simulink model "fft_biplex_real_4x_dsp48_opt_test"  (Simulink 7.4)
settings: Solver=VariableStepDiscrete  StartTime=0.0  StopTime=128  RelTol=1e-3
libraries: xbsIndex_r4 x620, casper_library_misc x24, casper_library_delays x6, casper_library_ffts_twiddle x1, simulink x1
(part 6 of 7)

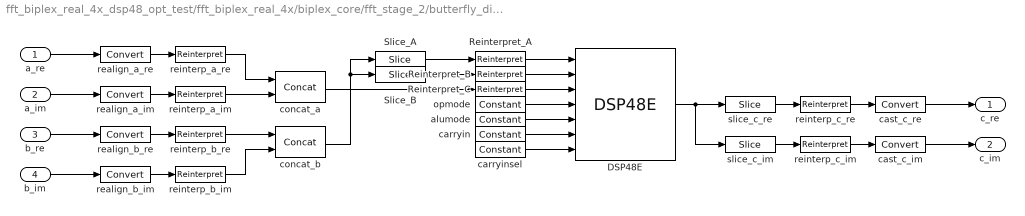
== system fft_biplex_real_4x_dsp48_opt_test/fft_biplex_real_4x/biplex_core/fft_stage_2/butterfly_direct/cadd ==
  a_re : Inport  OutDataType=sfix(16)  OutScaling=2^0
  a_im : Inport  Port=2  OutDataType=sfix(16)  OutScaling=2^0
  b_re : Inport  Port=3  OutDataType=sfix(16)  OutScaling=2^0
  b_im : Inport  Port=4  OutDataType=sfix(16)  OutScaling=2^0
  DSP48E : xbsIndex_r4/DSP48E  use_a=Direct from A Port  use_b=Direct from B Port  pattern_from_creg=off  pattern='000000000000'  mask_from_creg=off  pattern_mask='3FFFFFFFFFFF'  reset_preg=off  sel_rounding_mask=Select mask  use_op=off  use_creg=on  rst_all=off  en_all=off  use_pcin=off  use_carrycascin=off  use_multsignin=off  use_carryout=off  use_patterndetect=off  use_patternbdetect=off  use_overflow=off  use_underflow=off  use_acout=off  use_bcout=off  use_pcout=off  use_multsignout=off  use_carrycascout=off  pipeline_a=1  pipeline_b=1  pipeline_acout=1  pipeline_bcout=1  pipeline_c=on  pipeline_p=on  pipeline_mult=on  pipeline_opmode=on  pipeline_alumode=on  pipeline_carryin=on  pipeline_carryinsel=on  rst_a=off  rst_b=off  rst_c=off  rst_mult=off  rst_p=off  rst_carry_in=off  rst_alumode=off  rst_ctrl=off  en_a1=off  en_a2=off  en_b1=off  en_b2=off  en_c=off  en_mult=off  en_p=off  en_carry_in=off  en_alumode=off  en_multcarryin=off  en_ctrl=off  use_synth_model=off  addsub_mode=TWO24  xl_useadderonly=off  block_type=dsp48e
      settings: block_version=10.1.3
  Reinterpret_A : xbsIndex_r4/Reinterpret  force_arith_type=on  arith_type="Signed  (2's comp)"  force_bin_pt=on  bin_pt=0  block_type=reinterpret
      settings: infoedit="Changes signal type without altering the binary representation.   You can changed the signal between signed and unsigned, and relocate the binary point.<br><br>Hardware notes: In hardware this block costs nothing.<br><br>Example:  Suppose the input is 6 bits wide, signed, with 2 fractional bits, and the output is forced to unsigned with 0 fractional bits.  Then an input of -2.0 (1110.00 in binary 2's complement) becomes an output of 56 (111000 in binary)."  block_version=10.1.3
  Reinterpret_B : xbsIndex_r4/Reinterpret  force_arith_type=on  arith_type="Signed  (2's comp)"  force_bin_pt=on  bin_pt=0  block_type=reinterpret
      settings: infoedit="Changes signal type without altering the binary representation.   You can changed the signal between signed and unsigned, and relocate the binary point.<br><br>Hardware notes: In hardware this block costs nothing.<br><br>Example:  Suppose the input is 6 bits wide, signed, with 2 fractional bits, and the output is forced to unsigned with 0 fractional bits.  Then an input of -2.0 (1110.00 in binary 2's complement) becomes an output of 56 (111000 in binary)."  block_version=10.1.3
  Reinterpret_C : xbsIndex_r4/Reinterpret  force_arith_type=on  arith_type="Signed  (2's comp)"  force_bin_pt=on  bin_pt=0  block_type=reinterpret
      settings: infoedit="Changes signal type without altering the binary representation.   You can changed the signal between signed and unsigned, and relocate the binary point.<br><br>Hardware notes: In hardware this block costs nothing.<br><br>Example:  Suppose the input is 6 bits wide, signed, with 2 fractional bits, and the output is forced to unsigned with 0 fractional bits.  Then an input of -2.0 (1110.00 in binary 2's complement) becomes an output of 56 (111000 in binary)."  block_version=10.1.3
  Slice_A : xbsIndex_r4/Slice  nbits=30  boolean_output=off  mode=Upper Bit Location + Width  bit1=0  base1=MSB of Input  bit0=0  base0=LSB of Input  dbl_ovrd=off  block_type=slice
  Slice_B : xbsIndex_r4/Slice  nbits=18  boolean_output=off  mode=Lower Bit Location + Width  bit1=0  base1=MSB of Input  bit0=0  base0=LSB of Input  dbl_ovrd=off  block_type=slice
  alumode : xbsIndex_r4/Constant  arith_type=Unsigned  const=0  n_bits=4  bin_pt=0  explicit_period=off  period=1  equ=P=C  opselect=C  inp2=PCIN>>17  opr=+  inp1=P  carry=CIN  dbl_ovrd=off  block_type=constant
  carryin : xbsIndex_r4/Constant  arith_type=Unsigned  const=0  n_bits=1  bin_pt=0  explicit_period=off  period=1  equ=P=C  opselect=C  inp2=PCIN>>17  opr=+  inp1=P  carry=CIN  dbl_ovrd=off  block_type=constant
  carryinsel : xbsIndex_r4/Constant  arith_type=Unsigned  const=0  n_bits=3  bin_pt=0  explicit_period=off  period=1  equ=P=C  opselect=C  inp2=PCIN>>17  opr=+  inp1=P  carry=CIN  dbl_ovrd=off  block_type=constant
  cast_c_im : xbsIndex_r4/Convert  arith_type="Signed  (2's comp)"  n_bits=9  bin_pt=7  quantization=Truncate  overflow=Wrap  latency=0  dbl_ovrd=off  pipeline=on  block_type=convert
      settings: block_version=10.1.3
  cast_c_re : xbsIndex_r4/Convert  arith_type="Signed  (2's comp)"  n_bits=9  bin_pt=7  quantization=Truncate  overflow=Wrap  latency=0  dbl_ovrd=off  pipeline=on  block_type=convert
      settings: block_version=10.1.3
  concat_a : xbsIndex_r4/Concat  num_inputs=2  dbl_ovrd=off  block_type=concat
  concat_b : xbsIndex_r4/Concat  num_inputs=2  dbl_ovrd=off  block_type=concat
  opmode : xbsIndex_r4/Constant  arith_type=Unsigned  const=51  n_bits=7  bin_pt=0  explicit_period=off  period=1  equ=P=C  opselect=C  inp2=PCIN>>17  opr=+  inp1=P  carry=CIN  dbl_ovrd=off  block_type=constant
  realign_a_im : xbsIndex_r4/Convert  arith_type="Signed  (2's comp)"  n_bits=24  bin_pt=22  quantization=Truncate  overflow=Wrap  latency=0  dbl_ovrd=off  pipeline=on  block_type=convert
      settings: block_version=10.1.3
  realign_a_re : xbsIndex_r4/Convert  arith_type="Signed  (2's comp)"  n_bits=24  bin_pt=22  quantization=Truncate  overflow=Wrap  latency=0  dbl_ovrd=off  pipeline=on  block_type=convert
      settings: block_version=10.1.3
  realign_b_im : xbsIndex_r4/Convert  arith_type="Signed  (2's comp)"  n_bits=24  bin_pt=22  quantization=Truncate  overflow=Wrap  latency=0  dbl_ovrd=off  pipeline=on  block_type=convert
      settings: block_version=10.1.3
  realign_b_re : xbsIndex_r4/Convert  arith_type="Signed  (2's comp)"  n_bits=24  bin_pt=22  quantization=Truncate  overflow=Wrap  latency=0  dbl_ovrd=off  pipeline=on  block_type=convert
      settings: block_version=10.1.3
  reinterp_a_im : xbsIndex_r4/Reinterpret  force_arith_type=on  arith_type=Unsigned  force_bin_pt=on  bin_pt=0  block_type=reinterpret
      settings: infoedit="Changes signal type without altering the binary representation.   You can changed the signal between signed and unsigned, and relocate the binary point.<br><br>Hardware notes: In hardware this block costs nothing.<br><br>Example:  Suppose the input is 6 bits wide, signed, with 2 fractional bits, and the output is forced to unsigned with 0 fractional bits.  Then an input of -2.0 (1110.00 in binary 2's complement) becomes an output of 56 (111000 in binary)."  block_version=10.1.3
  reinterp_a_re : xbsIndex_r4/Reinterpret  force_arith_type=on  arith_type=Unsigned  force_bin_pt=on  bin_pt=0  block_type=reinterpret
      settings: infoedit="Changes signal type without altering the binary representation.   You can changed the signal between signed and unsigned, and relocate the binary point.<br><br>Hardware notes: In hardware this block costs nothing.<br><br>Example:  Suppose the input is 6 bits wide, signed, with 2 fractional bits, and the output is forced to unsigned with 0 fractional bits.  Then an input of -2.0 (1110.00 in binary 2's complement) becomes an output of 56 (111000 in binary)."  block_version=10.1.3
  reinterp_b_im : xbsIndex_r4/Reinterpret  force_arith_type=on  arith_type=Unsigned  force_bin_pt=on  bin_pt=0  block_type=reinterpret
      settings: infoedit="Changes signal type without altering the binary representation.   You can changed the signal between signed and unsigned, and relocate the binary point.<br><br>Hardware notes: In hardware this block costs nothing.<br><br>Example:  Suppose the input is 6 bits wide, signed, with 2 fractional bits, and the output is forced to unsigned with 0 fractional bits.  Then an input of -2.0 (1110.00 in binary 2's complement) becomes an output of 56 (111000 in binary)."  block_version=10.1.3
  reinterp_b_re : xbsIndex_r4/Reinterpret  force_arith_type=on  arith_type=Unsigned  force_bin_pt=on  bin_pt=0  block_type=reinterpret
      settings: infoedit="Changes signal type without altering the binary representation.   You can changed the signal between signed and unsigned, and relocate the binary point.<br><br>Hardware notes: In hardware this block costs nothing.<br><br>Example:  Suppose the input is 6 bits wide, signed, with 2 fractional bits, and the output is forced to unsigned with 0 fractional bits.  Then an input of -2.0 (1110.00 in binary 2's complement) becomes an output of 56 (111000 in binary)."  block_version=10.1.3
  reinterp_c_im : xbsIndex_r4/Reinterpret  force_arith_type=on  arith_type="Signed  (2's comp)"  force_bin_pt=on  bin_pt=22  block_type=reinterpret
      settings: infoedit="Changes signal type without altering the binary representation.   You can changed the signal between signed and unsigned, and relocate the binary point.<br><br>Hardware notes: In hardware this block costs nothing.<br><br>Example:  Suppose the input is 6 bits wide, signed, with 2 fractional bits, and the output is forced to unsigned with 0 fractional bits.  Then an input of -2.0 (1110.00 in binary 2's complement) becomes an output of 56 (111000 in binary)."  block_version=10.1.3
  reinterp_c_re : xbsIndex_r4/Reinterpret  force_arith_type=on  arith_type="Signed  (2's comp)"  force_bin_pt=on  bin_pt=22  block_type=reinterpret
      settings: infoedit="Changes signal type without altering the binary representation.   You can changed the signal between signed and unsigned, and relocate the binary point.<br><br>Hardware notes: In hardware this block costs nothing.<br><br>Example:  Suppose the input is 6 bits wide, signed, with 2 fractional bits, and the output is forced to unsigned with 0 fractional bits.  Then an input of -2.0 (1110.00 in binary 2's complement) becomes an output of 56 (111000 in binary)."  block_version=10.1.3
  slice_c_im : xbsIndex_r4/Slice  nbits=24  boolean_output=off  mode=Lower Bit Location + Width  bit1=0  base1=MSB of Input  bit0=0  base0=LSB of Input  dbl_ovrd=off  block_type=slice
  slice_c_re : xbsIndex_r4/Slice  nbits=24  boolean_output=off  mode=Lower Bit Location + Width  bit1=0  base1=MSB of Input  bit0=24  base0=LSB of Input  dbl_ovrd=off  block_type=slice
  c_re : Outport  OutDataType=sfix(16)  OutScaling=2^0
  c_im : Outport  Port=2  OutDataType=sfix(16)  OutScaling=2^0
  wires:
  realign_b_im/1 -> reinterp_b_im/1
  realign_b_re/1 -> reinterp_b_re/1
  realign_a_im/1 -> reinterp_a_im/1
  realign_a_re/1 -> reinterp_a_re/1
  a_re/1 -> realign_a_re/1
  b_re/1 -> realign_b_re/1
  Reinterpret_A/1 -> DSP48E/1
  Reinterpret_B/1 -> DSP48E/2
  opmode/1 -> DSP48E/4
  alumode/1 -> DSP48E/5
  carryin/1 -> DSP48E/6
  carryinsel/1 -> DSP48E/7
  a_im/1 -> realign_a_im/1
  b_im/1 -> realign_b_im/1
  concat_a/1 -> Reinterpret_C/1
  Slice_B/1 -> Reinterpret_B/1
  Slice_A/1 -> Reinterpret_A/1
  DSP48E/1 -> slice_c_re/1, slice_c_im/1
  slice_c_re/1 -> reinterp_c_re/1
  slice_c_im/1 -> reinterp_c_im/1
  reinterp_c_re/1 -> cast_c_re/1
  reinterp_c_im/1 -> cast_c_im/1
  Reinterpret_C/1 -> DSP48E/3
  concat_b/1 -> Slice_A/1, Slice_B/1
  reinterp_a_im/1 -> concat_a/2
  reinterp_b_re/1 -> concat_b/1
  reinterp_b_im/1 -> concat_b/2
  reinterp_a_re/1 -> concat_a/1
  cast_c_re/1 -> c_re/1
  cast_c_im/1 -> c_im/1

== system fft_biplex_real_4x_dsp48_opt_test/fft_biplex_real_4x/biplex_core/fft_stage_2/butterfly_direct/convert_of0 ==
  din : Inport  OutDataType=sfix(16)  OutScaling=2^0
  all_0s : xbsIndex_r4/Logical  logical_function=NAND  inputs=2  en=off  latency=latency  precision=Full  arith_type=Unsigned  n_bits=16  bin_pt=0  align_bp=on  dbl_ovrd=off  block_type=logical
  all_1s : xbsIndex_r4/Logical  logical_function=NAND  inputs=2  en=off  latency=latency  precision=Full  arith_type=Unsigned  n_bits=16  bin_pt=0  align_bp=on  dbl_ovrd=off  block_type=logical
  and : xbsIndex_r4/Logical  logical_function=AND  inputs=2  en=off  latency=0  precision=Full  arith_type=Unsigned  n_bits=16  bin_pt=0  align_bp=on  dbl_ovrd=off  block_type=logical
  convert : xbsIndex_r4/Convert  arith_type="Signed  (2's comp)"  n_bits=bit_width_o  bin_pt=binary_point_o  quantization=Truncate  overflow=Wrap  latency=latency  dbl_ovrd=off  pipeline=on  block_type=convert
      settings: block_version=10.1.1
  invert1 : xbsIndex_r4/Inverter  en=off  latency=0  dbl_ovrd=off  block_type=inv
  invert2 : xbsIndex_r4/Inverter  en=off  latency=0  dbl_ovrd=off  block_type=inv
  slice1 : xbsIndex_r4/Slice  nbits=1  boolean_output=on  mode=Upper Bit Location + Width  bit1=0  base1=MSB of Input  bit0=0  base0=LSB of Input  dbl_ovrd=off  block_type=slice
      settings: infoedit="Extracts a given range of bits from each input sample and presents it at the output.  The output type is ordinarily unsigned with binary point at zero, but can be Boolean when the slice is one bit wide.<P><P>Hardware notes: In hardware this block costs nothing."  block_version=10.1.1
  slice2 : xbsIndex_r4/Slice  nbits=1  boolean_output=on  mode=Upper Bit Location + Width  bit1=-1  base1=MSB of Input  bit0=0  base0=LSB of Input  dbl_ovrd=off  block_type=slice
      settings: infoedit="Extracts a given range of bits from each input sample and presents it at the output.  The output type is ordinarily unsigned with binary point at zero, but can be Boolean when the slice is one bit wide.<P><P>Hardware notes: In hardware this block costs nothing."  block_version=10.1.1
  dout : Outport
  of : Outport  Port=2
  wires:
  din/1 -> convert/1, slice1/1, slice2/1
  convert/1 -> dout/1
  slice1/1 -> all_1s/1, invert1/1
  invert1/1 -> all_0s/1
  slice2/1 -> all_1s/2, invert2/1
  invert2/1 -> all_0s/2
  all_0s/1 -> and/1
  all_1s/1 -> and/2
  and/1 -> of/1

== system fft_biplex_real_4x_dsp48_opt_test/fft_biplex_real_4x/biplex_core/fft_stage_2/butterfly_direct/convert_of1 ==
  din : Inport  OutDataType=sfix(16)  OutScaling=2^0
  all_0s : xbsIndex_r4/Logical  logical_function=NAND  inputs=2  en=off  latency=latency  precision=Full  arith_type=Unsigned  n_bits=16  bin_pt=0  align_bp=on  dbl_ovrd=off  block_type=logical
  all_1s : xbsIndex_r4/Logical  logical_function=NAND  inputs=2  en=off  latency=latency  precision=Full  arith_type=Unsigned  n_bits=16  bin_pt=0  align_bp=on  dbl_ovrd=off  block_type=logical
  and : xbsIndex_r4/Logical  logical_function=AND  inputs=2  en=off  latency=0  precision=Full  arith_type=Unsigned  n_bits=16  bin_pt=0  align_bp=on  dbl_ovrd=off  block_type=logical
  convert : xbsIndex_r4/Convert  arith_type="Signed  (2's comp)"  n_bits=bit_width_o  bin_pt=binary_point_o  quantization=Truncate  overflow=Wrap  latency=latency  dbl_ovrd=off  pipeline=on  block_type=convert
      settings: block_version=10.1.1
  invert1 : xbsIndex_r4/Inverter  en=off  latency=0  dbl_ovrd=off  block_type=inv
  invert2 : xbsIndex_r4/Inverter  en=off  latency=0  dbl_ovrd=off  block_type=inv
  slice1 : xbsIndex_r4/Slice  nbits=1  boolean_output=on  mode=Upper Bit Location + Width  bit1=0  base1=MSB of Input  bit0=0  base0=LSB of Input  dbl_ovrd=off  block_type=slice
      settings: infoedit="Extracts a given range of bits from each input sample and presents it at the output.  The output type is ordinarily unsigned with binary point at zero, but can be Boolean when the slice is one bit wide.<P><P>Hardware notes: In hardware this block costs nothing."  block_version=10.1.1
  slice2 : xbsIndex_r4/Slice  nbits=1  boolean_output=on  mode=Upper Bit Location + Width  bit1=-1  base1=MSB of Input  bit0=0  base0=LSB of Input  dbl_ovrd=off  block_type=slice
      settings: infoedit="Extracts a given range of bits from each input sample and presents it at the output.  The output type is ordinarily unsigned with binary point at zero, but can be Boolean when the slice is one bit wide.<P><P>Hardware notes: In hardware this block costs nothing."  block_version=10.1.1
  dout : Outport
  of : Outport  Port=2
  wires:
  din/1 -> convert/1, slice1/1, slice2/1
  convert/1 -> dout/1
  slice1/1 -> all_1s/1, invert1/1
  invert1/1 -> all_0s/1
  slice2/1 -> all_1s/2, invert2/1
  invert2/1 -> all_0s/2
  all_0s/1 -> and/1
  all_1s/1 -> and/2
  and/1 -> of/1

== system fft_biplex_real_4x_dsp48_opt_test/fft_biplex_real_4x/biplex_core/fft_stage_2/butterfly_direct/convert_of2 ==
  din : Inport  OutDataType=sfix(16)  OutScaling=2^0
  all_0s : xbsIndex_r4/Logical  logical_function=NAND  inputs=2  en=off  latency=latency  precision=Full  arith_type=Unsigned  n_bits=16  bin_pt=0  align_bp=on  dbl_ovrd=off  block_type=logical
  all_1s : xbsIndex_r4/Logical  logical_function=NAND  inputs=2  en=off  latency=latency  precision=Full  arith_type=Unsigned  n_bits=16  bin_pt=0  align_bp=on  dbl_ovrd=off  block_type=logical
  and : xbsIndex_r4/Logical  logical_function=AND  inputs=2  en=off  latency=0  precision=Full  arith_type=Unsigned  n_bits=16  bin_pt=0  align_bp=on  dbl_ovrd=off  block_type=logical
  convert : xbsIndex_r4/Convert  arith_type="Signed  (2's comp)"  n_bits=bit_width_o  bin_pt=binary_point_o  quantization=Truncate  overflow=Wrap  latency=latency  dbl_ovrd=off  pipeline=on  block_type=convert
      settings: block_version=10.1.1
  invert1 : xbsIndex_r4/Inverter  en=off  latency=0  dbl_ovrd=off  block_type=inv
  invert2 : xbsIndex_r4/Inverter  en=off  latency=0  dbl_ovrd=off  block_type=inv
  slice1 : xbsIndex_r4/Slice  nbits=1  boolean_output=on  mode=Upper Bit Location + Width  bit1=0  base1=MSB of Input  bit0=0  base0=LSB of Input  dbl_ovrd=off  block_type=slice
      settings: infoedit="Extracts a given range of bits from each input sample and presents it at the output.  The output type is ordinarily unsigned with binary point at zero, but can be Boolean when the slice is one bit wide.<P><P>Hardware notes: In hardware this block costs nothing."  block_version=10.1.1
  slice2 : xbsIndex_r4/Slice  nbits=1  boolean_output=on  mode=Upper Bit Location + Width  bit1=-1  base1=MSB of Input  bit0=0  base0=LSB of Input  dbl_ovrd=off  block_type=slice
      settings: infoedit="Extracts a given range of bits from each input sample and presents it at the output.  The output type is ordinarily unsigned with binary point at zero, but can be Boolean when the slice is one bit wide.<P><P>Hardware notes: In hardware this block costs nothing."  block_version=10.1.1
  dout : Outport
  of : Outport  Port=2
  wires:
  din/1 -> convert/1, slice1/1, slice2/1
  convert/1 -> dout/1
  slice1/1 -> all_1s/1, invert1/1
  invert1/1 -> all_0s/1
  slice2/1 -> all_1s/2, invert2/1
  invert2/1 -> all_0s/2
  all_0s/1 -> and/1
  all_1s/1 -> and/2
  and/1 -> of/1

== system fft_biplex_real_4x_dsp48_opt_test/fft_biplex_real_4x/biplex_core/fft_stage_2/butterfly_direct/convert_of3 ==
  din : Inport  OutDataType=sfix(16)  OutScaling=2^0
  all_0s : xbsIndex_r4/Logical  logical_function=NAND  inputs=2  en=off  latency=latency  precision=Full  arith_type=Unsigned  n_bits=16  bin_pt=0  align_bp=on  dbl_ovrd=off  block_type=logical
  all_1s : xbsIndex_r4/Logical  logical_function=NAND  inputs=2  en=off  latency=latency  precision=Full  arith_type=Unsigned  n_bits=16  bin_pt=0  align_bp=on  dbl_ovrd=off  block_type=logical
  and : xbsIndex_r4/Logical  logical_function=AND  inputs=2  en=off  latency=0  precision=Full  arith_type=Unsigned  n_bits=16  bin_pt=0  align_bp=on  dbl_ovrd=off  block_type=logical
  convert : xbsIndex_r4/Convert  arith_type="Signed  (2's comp)"  n_bits=bit_width_o  bin_pt=binary_point_o  quantization=Truncate  overflow=Wrap  latency=latency  dbl_ovrd=off  pipeline=on  block_type=convert
      settings: block_version=10.1.1
  invert1 : xbsIndex_r4/Inverter  en=off  latency=0  dbl_ovrd=off  block_type=inv
  invert2 : xbsIndex_r4/Inverter  en=off  latency=0  dbl_ovrd=off  block_type=inv
  slice1 : xbsIndex_r4/Slice  nbits=1  boolean_output=on  mode=Upper Bit Location + Width  bit1=0  base1=MSB of Input  bit0=0  base0=LSB of Input  dbl_ovrd=off  block_type=slice
      settings: infoedit="Extracts a given range of bits from each input sample and presents it at the output.  The output type is ordinarily unsigned with binary point at zero, but can be Boolean when the slice is one bit wide.<P><P>Hardware notes: In hardware this block costs nothing."  block_version=10.1.1
  slice2 : xbsIndex_r4/Slice  nbits=1  boolean_output=on  mode=Upper Bit Location + Width  bit1=-1  base1=MSB of Input  bit0=0  base0=LSB of Input  dbl_ovrd=off  block_type=slice
      settings: infoedit="Extracts a given range of bits from each input sample and presents it at the output.  The output type is ordinarily unsigned with binary point at zero, but can be Boolean when the slice is one bit wide.<P><P>Hardware notes: In hardware this block costs nothing."  block_version=10.1.1
  dout : Outport
  of : Outport  Port=2
  wires:
  din/1 -> convert/1, slice1/1, slice2/1
  convert/1 -> dout/1
  slice1/1 -> all_1s/1, invert1/1
  invert1/1 -> all_0s/1
  slice2/1 -> all_1s/2, invert2/1
  invert2/1 -> all_0s/2
  all_0s/1 -> and/1
  all_1s/1 -> and/2
  and/1 -> of/1

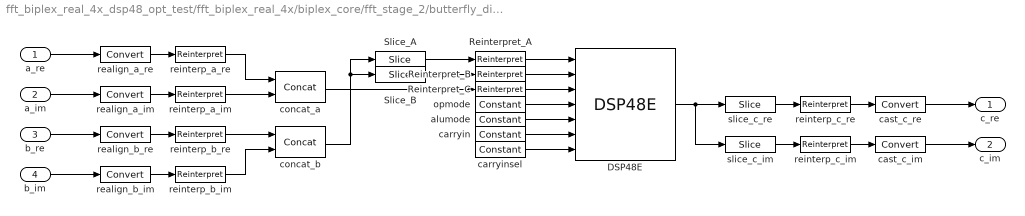
== system fft_biplex_real_4x_dsp48_opt_test/fft_biplex_real_4x/biplex_core/fft_stage_2/butterfly_direct/csub ==
  a_re : Inport  OutDataType=sfix(16)  OutScaling=2^0
  a_im : Inport  Port=2  OutDataType=sfix(16)  OutScaling=2^0
  b_re : Inport  Port=3  OutDataType=sfix(16)  OutScaling=2^0
  b_im : Inport  Port=4  OutDataType=sfix(16)  OutScaling=2^0
  DSP48E : xbsIndex_r4/DSP48E  use_a=Direct from A Port  use_b=Direct from B Port  pattern_from_creg=off  pattern='000000000000'  mask_from_creg=off  pattern_mask='3FFFFFFFFFFF'  reset_preg=off  sel_rounding_mask=Select mask  use_op=off  use_creg=on  rst_all=off  en_all=off  use_pcin=off  use_carrycascin=off  use_multsignin=off  use_carryout=off  use_patterndetect=off  use_patternbdetect=off  use_overflow=off  use_underflow=off  use_acout=off  use_bcout=off  use_pcout=off  use_multsignout=off  use_carrycascout=off  pipeline_a=1  pipeline_b=1  pipeline_acout=1  pipeline_bcout=1  pipeline_c=on  pipeline_p=on  pipeline_mult=on  pipeline_opmode=on  pipeline_alumode=on  pipeline_carryin=on  pipeline_carryinsel=on  rst_a=off  rst_b=off  rst_c=off  rst_mult=off  rst_p=off  rst_carry_in=off  rst_alumode=off  rst_ctrl=off  en_a1=off  en_a2=off  en_b1=off  en_b2=off  en_c=off  en_mult=off  en_p=off  en_carry_in=off  en_alumode=off  en_multcarryin=off  en_ctrl=off  use_synth_model=off  addsub_mode=TWO24  xl_useadderonly=off  block_type=dsp48e
      settings: block_version=10.1.3
  Reinterpret_A : xbsIndex_r4/Reinterpret  force_arith_type=on  arith_type="Signed  (2's comp)"  force_bin_pt=on  bin_pt=0  block_type=reinterpret
      settings: infoedit="Changes signal type without altering the binary representation.   You can changed the signal between signed and unsigned, and relocate the binary point.<br><br>Hardware notes: In hardware this block costs nothing.<br><br>Example:  Suppose the input is 6 bits wide, signed, with 2 fractional bits, and the output is forced to unsigned with 0 fractional bits.  Then an input of -2.0 (1110.00 in binary 2's complement) becomes an output of 56 (111000 in binary)."  block_version=10.1.3
  Reinterpret_B : xbsIndex_r4/Reinterpret  force_arith_type=on  arith_type="Signed  (2's comp)"  force_bin_pt=on  bin_pt=0  block_type=reinterpret
      settings: infoedit="Changes signal type without altering the binary representation.   You can changed the signal between signed and unsigned, and relocate the binary point.<br><br>Hardware notes: In hardware this block costs nothing.<br><br>Example:  Suppose the input is 6 bits wide, signed, with 2 fractional bits, and the output is forced to unsigned with 0 fractional bits.  Then an input of -2.0 (1110.00 in binary 2's complement) becomes an output of 56 (111000 in binary)."  block_version=10.1.3
  Reinterpret_C : xbsIndex_r4/Reinterpret  force_arith_type=on  arith_type="Signed  (2's comp)"  force_bin_pt=on  bin_pt=0  block_type=reinterpret
      settings: infoedit="Changes signal type without altering the binary representation.   You can changed the signal between signed and unsigned, and relocate the binary point.<br><br>Hardware notes: In hardware this block costs nothing.<br><br>Example:  Suppose the input is 6 bits wide, signed, with 2 fractional bits, and the output is forced to unsigned with 0 fractional bits.  Then an input of -2.0 (1110.00 in binary 2's complement) becomes an output of 56 (111000 in binary)."  block_version=10.1.3
  Slice_A : xbsIndex_r4/Slice  nbits=30  boolean_output=off  mode=Upper Bit Location + Width  bit1=0  base1=MSB of Input  bit0=0  base0=LSB of Input  dbl_ovrd=off  block_type=slice
  Slice_B : xbsIndex_r4/Slice  nbits=18  boolean_output=off  mode=Lower Bit Location + Width  bit1=0  base1=MSB of Input  bit0=0  base0=LSB of Input  dbl_ovrd=off  block_type=slice
  alumode : xbsIndex_r4/Constant  arith_type=Unsigned  const=3  n_bits=4  bin_pt=0  explicit_period=off  period=1  equ=P=C  opselect=C  inp2=PCIN>>17  opr=+  inp1=P  carry=CIN  dbl_ovrd=off  block_type=constant
  carryin : xbsIndex_r4/Constant  arith_type=Unsigned  const=0  n_bits=1  bin_pt=0  explicit_period=off  period=1  equ=P=C  opselect=C  inp2=PCIN>>17  opr=+  inp1=P  carry=CIN  dbl_ovrd=off  block_type=constant
  carryinsel : xbsIndex_r4/Constant  arith_type=Unsigned  const=0  n_bits=3  bin_pt=0  explicit_period=off  period=1  equ=P=C  opselect=C  inp2=PCIN>>17  opr=+  inp1=P  carry=CIN  dbl_ovrd=off  block_type=constant
  cast_c_im : xbsIndex_r4/Convert  arith_type="Signed  (2's comp)"  n_bits=9  bin_pt=7  quantization=Truncate  overflow=Wrap  latency=0  dbl_ovrd=off  pipeline=on  block_type=convert
      settings: block_version=10.1.3
  cast_c_re : xbsIndex_r4/Convert  arith_type="Signed  (2's comp)"  n_bits=9  bin_pt=7  quantization=Truncate  overflow=Wrap  latency=0  dbl_ovrd=off  pipeline=on  block_type=convert
      settings: block_version=10.1.3
  concat_a : xbsIndex_r4/Concat  num_inputs=2  dbl_ovrd=off  block_type=concat
  concat_b : xbsIndex_r4/Concat  num_inputs=2  dbl_ovrd=off  block_type=concat
  opmode : xbsIndex_r4/Constant  arith_type=Unsigned  const=51  n_bits=7  bin_pt=0  explicit_period=off  period=1  equ=P=C  opselect=C  inp2=PCIN>>17  opr=+  inp1=P  carry=CIN  dbl_ovrd=off  block_type=constant
  realign_a_im : xbsIndex_r4/Convert  arith_type="Signed  (2's comp)"  n_bits=24  bin_pt=22  quantization=Truncate  overflow=Wrap  latency=0  dbl_ovrd=off  pipeline=on  block_type=convert
      settings: block_version=10.1.3
  realign_a_re : xbsIndex_r4/Convert  arith_type="Signed  (2's comp)"  n_bits=24  bin_pt=22  quantization=Truncate  overflow=Wrap  latency=0  dbl_ovrd=off  pipeline=on  block_type=convert
      settings: block_version=10.1.3
  realign_b_im : xbsIndex_r4/Convert  arith_type="Signed  (2's comp)"  n_bits=24  bin_pt=22  quantization=Truncate  overflow=Wrap  latency=0  dbl_ovrd=off  pipeline=on  block_type=convert
      settings: block_version=10.1.3
  realign_b_re : xbsIndex_r4/Convert  arith_type="Signed  (2's comp)"  n_bits=24  bin_pt=22  quantization=Truncate  overflow=Wrap  latency=0  dbl_ovrd=off  pipeline=on  block_type=convert
      settings: block_version=10.1.3
  reinterp_a_im : xbsIndex_r4/Reinterpret  force_arith_type=on  arith_type=Unsigned  force_bin_pt=on  bin_pt=0  block_type=reinterpret
      settings: infoedit="Changes signal type without altering the binary representation.   You can changed the signal between signed and unsigned, and relocate the binary point.<br><br>Hardware notes: In hardware this block costs nothing.<br><br>Example:  Suppose the input is 6 bits wide, signed, with 2 fractional bits, and the output is forced to unsigned with 0 fractional bits.  Then an input of -2.0 (1110.00 in binary 2's complement) becomes an output of 56 (111000 in binary)."  block_version=10.1.3
  reinterp_a_re : xbsIndex_r4/Reinterpret  force_arith_type=on  arith_type=Unsigned  force_bin_pt=on  bin_pt=0  block_type=reinterpret
      settings: infoedit="Changes signal type without altering the binary representation.   You can changed the signal between signed and unsigned, and relocate the binary point.<br><br>Hardware notes: In hardware this block costs nothing.<br><br>Example:  Suppose the input is 6 bits wide, signed, with 2 fractional bits, and the output is forced to unsigned with 0 fractional bits.  Then an input of -2.0 (1110.00 in binary 2's complement) becomes an output of 56 (111000 in binary)."  block_version=10.1.3
  reinterp_b_im : xbsIndex_r4/Reinterpret  force_arith_type=on  arith_type=Unsigned  force_bin_pt=on  bin_pt=0  block_type=reinterpret
      settings: infoedit="Changes signal type without altering the binary representation.   You can changed the signal between signed and unsigned, and relocate the binary point.<br><br>Hardware notes: In hardware this block costs nothing.<br><br>Example:  Suppose the input is 6 bits wide, signed, with 2 fractional bits, and the output is forced to unsigned with 0 fractional bits.  Then an input of -2.0 (1110.00 in binary 2's complement) becomes an output of 56 (111000 in binary)."  block_version=10.1.3
  reinterp_b_re : xbsIndex_r4/Reinterpret  force_arith_type=on  arith_type=Unsigned  force_bin_pt=on  bin_pt=0  block_type=reinterpret
      settings: infoedit="Changes signal type without altering the binary representation.   You can changed the signal between signed and unsigned, and relocate the binary point.<br><br>Hardware notes: In hardware this block costs nothing.<br><br>Example:  Suppose the input is 6 bits wide, signed, with 2 fractional bits, and the output is forced to unsigned with 0 fractional bits.  Then an input of -2.0 (1110.00 in binary 2's complement) becomes an output of 56 (111000 in binary)."  block_version=10.1.3
  reinterp_c_im : xbsIndex_r4/Reinterpret  force_arith_type=on  arith_type="Signed  (2's comp)"  force_bin_pt=on  bin_pt=22  block_type=reinterpret
      settings: infoedit="Changes signal type without altering the binary representation.   You can changed the signal between signed and unsigned, and relocate the binary point.<br><br>Hardware notes: In hardware this block costs nothing.<br><br>Example:  Suppose the input is 6 bits wide, signed, with 2 fractional bits, and the output is forced to unsigned with 0 fractional bits.  Then an input of -2.0 (1110.00 in binary 2's complement) becomes an output of 56 (111000 in binary)."  block_version=10.1.3
  reinterp_c_re : xbsIndex_r4/Reinterpret  force_arith_type=on  arith_type="Signed  (2's comp)"  force_bin_pt=on  bin_pt=22  block_type=reinterpret
      settings: infoedit="Changes signal type without altering the binary representation.   You can changed the signal between signed and unsigned, and relocate the binary point.<br><br>Hardware notes: In hardware this block costs nothing.<br><br>Example:  Suppose the input is 6 bits wide, signed, with 2 fractional bits, and the output is forced to unsigned with 0 fractional bits.  Then an input of -2.0 (1110.00 in binary 2's complement) becomes an output of 56 (111000 in binary)."  block_version=10.1.3
  slice_c_im : xbsIndex_r4/Slice  nbits=24  boolean_output=off  mode=Lower Bit Location + Width  bit1=0  base1=MSB of Input  bit0=0  base0=LSB of Input  dbl_ovrd=off  block_type=slice
  slice_c_re : xbsIndex_r4/Slice  nbits=24  boolean_output=off  mode=Lower Bit Location + Width  bit1=0  base1=MSB of Input  bit0=24  base0=LSB of Input  dbl_ovrd=off  block_type=slice
  c_re : Outport  OutDataType=sfix(16)  OutScaling=2^0
  c_im : Outport  Port=2  OutDataType=sfix(16)  OutScaling=2^0
  wires:
  realign_b_im/1 -> reinterp_b_im/1
  realign_b_re/1 -> reinterp_b_re/1
  realign_a_im/1 -> reinterp_a_im/1
  realign_a_re/1 -> reinterp_a_re/1
  a_re/1 -> realign_a_re/1
  b_re/1 -> realign_b_re/1
  Reinterpret_A/1 -> DSP48E/1
  Reinterpret_B/1 -> DSP48E/2
  opmode/1 -> DSP48E/4
  alumode/1 -> DSP48E/5
  carryin/1 -> DSP48E/6
  carryinsel/1 -> DSP48E/7
  a_im/1 -> realign_a_im/1
  b_im/1 -> realign_b_im/1
  concat_a/1 -> Reinterpret_C/1
  Slice_B/1 -> Reinterpret_B/1
  Slice_A/1 -> Reinterpret_A/1
  DSP48E/1 -> slice_c_re/1, slice_c_im/1
  slice_c_re/1 -> reinterp_c_re/1
  slice_c_im/1 -> reinterp_c_im/1
  reinterp_c_re/1 -> cast_c_re/1
  reinterp_c_im/1 -> cast_c_im/1
  Reinterpret_C/1 -> DSP48E/3
  concat_b/1 -> Slice_A/1, Slice_B/1
  reinterp_a_im/1 -> concat_a/2
  reinterp_b_re/1 -> concat_b/1
  reinterp_b_im/1 -> concat_b/2
  reinterp_a_re/1 -> concat_a/1
  cast_c_re/1 -> c_re/1
  cast_c_im/1 -> c_im/1

== system fft_biplex_real_4x_dsp48_opt_test/fft_biplex_real_4x/biplex_core/fft_stage_2/butterfly_direct/twiddle_stage_2 ==
  a : Inport  OutDataType=sfix(16)  OutScaling=2^0
  b : Inport  Port=2  OutDataType=sfix(16)  OutScaling=2^0
  sync : Inport  Port=3  OutDataType=sfix(16)  OutScaling=2^0
  c_to_ri : casper_library_misc/c_to_ri  SystemSampleTime=-1  n_bits=input_bit_width  bin_pt=input_bit_width-1
      settings: AttributesFormatString=8_7 r/i
  c_to_ri1 : casper_library_misc/c_to_ri  SystemSampleTime=-1  n_bits=input_bit_width  bin_pt=input_bit_width-1
      settings: AttributesFormatString=8_7 r/i
  counter : xbsIndex_r4/Counter  cnt_type=Free Running  cnt_to=Inf  operation=Up  start_count=0  cnt_by_val=1  arith_type=Unsigned  n_bits=FFTSize - 1  bin_pt=0  load_pin=off  rst=on  en=off  explicit_period=on  period=1  dbl_ovrd=off  use_behavioral_HDL=on  implementation=Fabric  block_type=counter
      settings: block_version=11.4
  delay0 : xbsIndex_r4/Delay  en=off  latency=bram_latency+mult_latency+conv_latency+add_latency  dbl_ovrd=off  reg_retiming=on  block_type=delay
      settings: block_version=11.4
  delay1 : xbsIndex_r4/Delay  en=off  latency=bram_latency+mult_latency+conv_latency+add_latency  dbl_ovrd=off  reg_retiming=on  block_type=delay
      settings: block_version=11.4
  delay2 : xbsIndex_r4/Delay  en=off  latency=bram_latency  dbl_ovrd=off  reg_retiming=on  block_type=delay
      settings: block_version=11.4
  delay5 : xbsIndex_r4/Delay  en=off  latency=bram_latency  dbl_ovrd=off  reg_retiming=on  block_type=delay
      settings: block_version=11.4
  delay6 : xbsIndex_r4/Delay  en=off  latency=mult_latency+conv_latency+add_latency  dbl_ovrd=off  reg_retiming=on  block_type=delay
      settings: block_version=11.4
  delay7 : xbsIndex_r4/Delay  en=off  latency=bram_latency  dbl_ovrd=off  reg_retiming=on  block_type=delay
      settings: block_version=11.4
  mux0 : xbsIndex_r4/Mux  inputs=2  en=off  latency=6  precision=Full  arith_type=Unsigned  n_bits=16  bin_pt=14  quantization=Truncate  overflow=Wrap  dbl_ovrd=off  block_type=mux
      settings: block_version=11.4
  mux1 : xbsIndex_r4/Mux  inputs=2  en=off  latency=6  precision=Full  arith_type=Unsigned  n_bits=16  bin_pt=14  quantization=Truncate  overflow=Wrap  dbl_ovrd=off  block_type=mux
      settings: block_version=11.4
  negate : xbsIndex_r4/Negate  precision=User Defined  arith_type="Signed  (2's comp)"  n_bits=input_bit_width  bin_pt=input_bit_width-1  quantization=Truncate  overflow=Saturate  en=off  latency=bram_latency  dbl_ovrd=off  block_type=negate
      settings: block_version=11.4
  slice : xbsIndex_r4/Slice  nbits=1  boolean_output=off  mode=Upper Bit Location + Width  bit1=0  base1=MSB of Input  bit0=0  base0=LSB of Input  dbl_ovrd=off  block_type=slice
  a_re : Outport  OutDataType=sfix(16)  OutScaling=2^0
  a_im : Outport  Port=2  OutDataType=sfix(16)  OutScaling=2^0
  bw_re : Outport  Port=3  OutDataType=sfix(16)  OutScaling=2^0
  bw_im : Outport  Port=4  OutDataType=sfix(16)  OutScaling=2^0
  sync_out : Outport  Port=5  OutDataType=sfix(16)  OutScaling=2^0
  wires:
  negate/1 -> mux1/3
  delay7/1 -> mux0/3, mux1/2
  c_to_ri1/2 -> delay7/1
  delay6/1 -> sync_out/1
  delay5/1 -> counter/1, delay6/1
  sync/1 -> delay5/1
  mux1/1 -> bw_im/1
  mux0/1 -> bw_re/1
  slice/1 -> mux0/1, mux1/1
  counter/1 -> slice/1
  delay2/1 -> mux0/2
  c_to_ri1/1 -> negate/1, delay2/1
  delay1/1 -> a_im/1
  delay0/1 -> a_re/1
  c_to_ri/2 -> delay1/1
  c_to_ri/1 -> delay0/1
  b/1 -> c_to_ri1/1
  a/1 -> c_to_ri/1

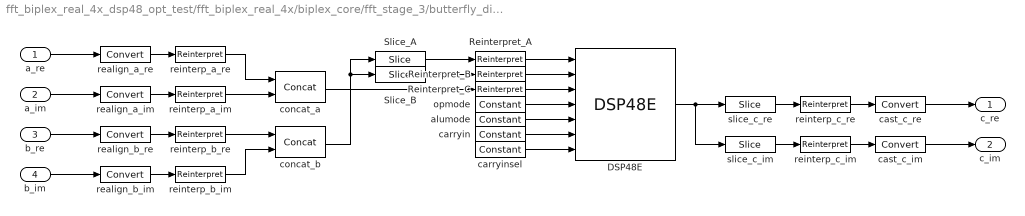
== system fft_biplex_real_4x_dsp48_opt_test/fft_biplex_real_4x/biplex_core/fft_stage_3/butterfly_direct/cadd ==
  a_re : Inport  OutDataType=sfix(16)  OutScaling=2^0
  a_im : Inport  Port=2  OutDataType=sfix(16)  OutScaling=2^0
  b_re : Inport  Port=3  OutDataType=sfix(16)  OutScaling=2^0
  b_im : Inport  Port=4  OutDataType=sfix(16)  OutScaling=2^0
  DSP48E : xbsIndex_r4/DSP48E  use_a=Direct from A Port  use_b=Direct from B Port  pattern_from_creg=off  pattern='000000000000'  mask_from_creg=off  pattern_mask='3FFFFFFFFFFF'  reset_preg=off  sel_rounding_mask=Select mask  use_op=off  use_creg=on  rst_all=off  en_all=off  use_pcin=off  use_carrycascin=off  use_multsignin=off  use_carryout=off  use_patterndetect=off  use_patternbdetect=off  use_overflow=off  use_underflow=off  use_acout=off  use_bcout=off  use_pcout=off  use_multsignout=off  use_carrycascout=off  pipeline_a=1  pipeline_b=1  pipeline_acout=1  pipeline_bcout=1  pipeline_c=on  pipeline_p=on  pipeline_mult=on  pipeline_opmode=on  pipeline_alumode=on  pipeline_carryin=on  pipeline_carryinsel=on  rst_a=off  rst_b=off  rst_c=off  rst_mult=off  rst_p=off  rst_carry_in=off  rst_alumode=off  rst_ctrl=off  en_a1=off  en_a2=off  en_b1=off  en_b2=off  en_c=off  en_mult=off  en_p=off  en_carry_in=off  en_alumode=off  en_multcarryin=off  en_ctrl=off  use_synth_model=off  addsub_mode=TWO24  xl_useadderonly=off  block_type=dsp48e
      settings: block_version=10.1.3
  Reinterpret_A : xbsIndex_r4/Reinterpret  force_arith_type=on  arith_type="Signed  (2's comp)"  force_bin_pt=on  bin_pt=0  block_type=reinterpret
      settings: infoedit="Changes signal type without altering the binary representation.   You can changed the signal between signed and unsigned, and relocate the binary point.<br><br>Hardware notes: In hardware this block costs nothing.<br><br>Example:  Suppose the input is 6 bits wide, signed, with 2 fractional bits, and the output is forced to unsigned with 0 fractional bits.  Then an input of -2.0 (1110.00 in binary 2's complement) becomes an output of 56 (111000 in binary)."  block_version=10.1.3
  Reinterpret_B : xbsIndex_r4/Reinterpret  force_arith_type=on  arith_type="Signed  (2's comp)"  force_bin_pt=on  bin_pt=0  block_type=reinterpret
      settings: infoedit="Changes signal type without altering the binary representation.   You can changed the signal between signed and unsigned, and relocate the binary point.<br><br>Hardware notes: In hardware this block costs nothing.<br><br>Example:  Suppose the input is 6 bits wide, signed, with 2 fractional bits, and the output is forced to unsigned with 0 fractional bits.  Then an input of -2.0 (1110.00 in binary 2's complement) becomes an output of 56 (111000 in binary)."  block_version=10.1.3
  Reinterpret_C : xbsIndex_r4/Reinterpret  force_arith_type=on  arith_type="Signed  (2's comp)"  force_bin_pt=on  bin_pt=0  block_type=reinterpret
      settings: infoedit="Changes signal type without altering the binary representation.   You can changed the signal between signed and unsigned, and relocate the binary point.<br><br>Hardware notes: In hardware this block costs nothing.<br><br>Example:  Suppose the input is 6 bits wide, signed, with 2 fractional bits, and the output is forced to unsigned with 0 fractional bits.  Then an input of -2.0 (1110.00 in binary 2's complement) becomes an output of 56 (111000 in binary)."  block_version=10.1.3
  Slice_A : xbsIndex_r4/Slice  nbits=30  boolean_output=off  mode=Upper Bit Location + Width  bit1=0  base1=MSB of Input  bit0=0  base0=LSB of Input  dbl_ovrd=off  block_type=slice
  Slice_B : xbsIndex_r4/Slice  nbits=18  boolean_output=off  mode=Lower Bit Location + Width  bit1=0  base1=MSB of Input  bit0=0  base0=LSB of Input  dbl_ovrd=off  block_type=slice
  alumode : xbsIndex_r4/Constant  arith_type=Unsigned  const=0  n_bits=4  bin_pt=0  explicit_period=off  period=1  equ=P=C  opselect=C  inp2=PCIN>>17  opr=+  inp1=P  carry=CIN  dbl_ovrd=off  block_type=constant
  carryin : xbsIndex_r4/Constant  arith_type=Unsigned  const=0  n_bits=1  bin_pt=0  explicit_period=off  period=1  equ=P=C  opselect=C  inp2=PCIN>>17  opr=+  inp1=P  carry=CIN  dbl_ovrd=off  block_type=constant
  carryinsel : xbsIndex_r4/Constant  arith_type=Unsigned  const=0  n_bits=3  bin_pt=0  explicit_period=off  period=1  equ=P=C  opselect=C  inp2=PCIN>>17  opr=+  inp1=P  carry=CIN  dbl_ovrd=off  block_type=constant
  cast_c_im : xbsIndex_r4/Convert  arith_type="Signed  (2's comp)"  n_bits=13  bin_pt=9  quantization=Truncate  overflow=Wrap  latency=0  dbl_ovrd=off  pipeline=on  block_type=convert
      settings: block_version=10.1.3
  cast_c_re : xbsIndex_r4/Convert  arith_type="Signed  (2's comp)"  n_bits=13  bin_pt=9  quantization=Truncate  overflow=Wrap  latency=0  dbl_ovrd=off  pipeline=on  block_type=convert
      settings: block_version=10.1.3
  concat_a : xbsIndex_r4/Concat  num_inputs=2  dbl_ovrd=off  block_type=concat
  concat_b : xbsIndex_r4/Concat  num_inputs=2  dbl_ovrd=off  block_type=concat
  opmode : xbsIndex_r4/Constant  arith_type=Unsigned  const=51  n_bits=7  bin_pt=0  explicit_period=off  period=1  equ=P=C  opselect=C  inp2=PCIN>>17  opr=+  inp1=P  carry=CIN  dbl_ovrd=off  block_type=constant
  realign_a_im : xbsIndex_r4/Convert  arith_type="Signed  (2's comp)"  n_bits=24  bin_pt=20  quantization=Truncate  overflow=Wrap  latency=0  dbl_ovrd=off  pipeline=on  block_type=convert
      settings: block_version=10.1.3
  realign_a_re : xbsIndex_r4/Convert  arith_type="Signed  (2's comp)"  n_bits=24  bin_pt=20  quantization=Truncate  overflow=Wrap  latency=0  dbl_ovrd=off  pipeline=on  block_type=convert
      settings: block_version=10.1.3
  realign_b_im : xbsIndex_r4/Convert  arith_type="Signed  (2's comp)"  n_bits=24  bin_pt=20  quantization=Truncate  overflow=Wrap  latency=0  dbl_ovrd=off  pipeline=on  block_type=convert
      settings: block_version=10.1.3
  realign_b_re : xbsIndex_r4/Convert  arith_type="Signed  (2's comp)"  n_bits=24  bin_pt=20  quantization=Truncate  overflow=Wrap  latency=0  dbl_ovrd=off  pipeline=on  block_type=convert
      settings: block_version=10.1.3
  reinterp_a_im : xbsIndex_r4/Reinterpret  force_arith_type=on  arith_type=Unsigned  force_bin_pt=on  bin_pt=0  block_type=reinterpret
      settings: infoedit="Changes signal type without altering the binary representation.   You can changed the signal between signed and unsigned, and relocate the binary point.<br><br>Hardware notes: In hardware this block costs nothing.<br><br>Example:  Suppose the input is 6 bits wide, signed, with 2 fractional bits, and the output is forced to unsigned with 0 fractional bits.  Then an input of -2.0 (1110.00 in binary 2's complement) becomes an output of 56 (111000 in binary)."  block_version=10.1.3
  reinterp_a_re : xbsIndex_r4/Reinterpret  force_arith_type=on  arith_type=Unsigned  force_bin_pt=on  bin_pt=0  block_type=reinterpret
      settings: infoedit="Changes signal type without altering the binary representation.   You can changed the signal between signed and unsigned, and relocate the binary point.<br><br>Hardware notes: In hardware this block costs nothing.<br><br>Example:  Suppose the input is 6 bits wide, signed, with 2 fractional bits, and the output is forced to unsigned with 0 fractional bits.  Then an input of -2.0 (1110.00 in binary 2's complement) becomes an output of 56 (111000 in binary)."  block_version=10.1.3
  reinterp_b_im : xbsIndex_r4/Reinterpret  force_arith_type=on  arith_type=Unsigned  force_bin_pt=on  bin_pt=0  block_type=reinterpret
      settings: infoedit="Changes signal type without altering the binary representation.   You can changed the signal between signed and unsigned, and relocate the binary point.<br><br>Hardware notes: In hardware this block costs nothing.<br><br>Example:  Suppose the input is 6 bits wide, signed, with 2 fractional bits, and the output is forced to unsigned with 0 fractional bits.  Then an input of -2.0 (1110.00 in binary 2's complement) becomes an output of 56 (111000 in binary)."  block_version=10.1.3
  reinterp_b_re : xbsIndex_r4/Reinterpret  force_arith_type=on  arith_type=Unsigned  force_bin_pt=on  bin_pt=0  block_type=reinterpret
      settings: infoedit="Changes signal type without altering the binary representation.   You can changed the signal between signed and unsigned, and relocate the binary point.<br><br>Hardware notes: In hardware this block costs nothing.<br><br>Example:  Suppose the input is 6 bits wide, signed, with 2 fractional bits, and the output is forced to unsigned with 0 fractional bits.  Then an input of -2.0 (1110.00 in binary 2's complement) becomes an output of 56 (111000 in binary)."  block_version=10.1.3
  reinterp_c_im : xbsIndex_r4/Reinterpret  force_arith_type=on  arith_type="Signed  (2's comp)"  force_bin_pt=on  bin_pt=20  block_type=reinterpret
      settings: infoedit="Changes signal type without altering the binary representation.   You can changed the signal between signed and unsigned, and relocate the binary point.<br><br>Hardware notes: In hardware this block costs nothing.<br><br>Example:  Suppose the input is 6 bits wide, signed, with 2 fractional bits, and the output is forced to unsigned with 0 fractional bits.  Then an input of -2.0 (1110.00 in binary 2's complement) becomes an output of 56 (111000 in binary)."  block_version=10.1.3
  reinterp_c_re : xbsIndex_r4/Reinterpret  force_arith_type=on  arith_type="Signed  (2's comp)"  force_bin_pt=on  bin_pt=20  block_type=reinterpret
      settings: infoedit="Changes signal type without altering the binary representation.   You can changed the signal between signed and unsigned, and relocate the binary point.<br><br>Hardware notes: In hardware this block costs nothing.<br><br>Example:  Suppose the input is 6 bits wide, signed, with 2 fractional bits, and the output is forced to unsigned with 0 fractional bits.  Then an input of -2.0 (1110.00 in binary 2's complement) becomes an output of 56 (111000 in binary)."  block_version=10.1.3
  slice_c_im : xbsIndex_r4/Slice  nbits=24  boolean_output=off  mode=Lower Bit Location + Width  bit1=0  base1=MSB of Input  bit0=0  base0=LSB of Input  dbl_ovrd=off  block_type=slice
  slice_c_re : xbsIndex_r4/Slice  nbits=24  boolean_output=off  mode=Lower Bit Location + Width  bit1=0  base1=MSB of Input  bit0=24  base0=LSB of Input  dbl_ovrd=off  block_type=slice
  c_re : Outport  OutDataType=sfix(16)  OutScaling=2^0
  c_im : Outport  Port=2  OutDataType=sfix(16)  OutScaling=2^0
  wires:
  realign_b_im/1 -> reinterp_b_im/1
  realign_b_re/1 -> reinterp_b_re/1
  realign_a_im/1 -> reinterp_a_im/1
  realign_a_re/1 -> reinterp_a_re/1
  a_re/1 -> realign_a_re/1
  b_re/1 -> realign_b_re/1
  Reinterpret_A/1 -> DSP48E/1
  Reinterpret_B/1 -> DSP48E/2
  opmode/1 -> DSP48E/4
  alumode/1 -> DSP48E/5
  carryin/1 -> DSP48E/6
  carryinsel/1 -> DSP48E/7
  a_im/1 -> realign_a_im/1
  b_im/1 -> realign_b_im/1
  concat_a/1 -> Reinterpret_C/1
  Slice_B/1 -> Reinterpret_B/1
  Slice_A/1 -> Reinterpret_A/1
  DSP48E/1 -> slice_c_re/1, slice_c_im/1
  slice_c_re/1 -> reinterp_c_re/1
  slice_c_im/1 -> reinterp_c_im/1
  reinterp_c_re/1 -> cast_c_re/1
  reinterp_c_im/1 -> cast_c_im/1
  Reinterpret_C/1 -> DSP48E/3
  concat_b/1 -> Slice_A/1, Slice_B/1
  reinterp_a_im/1 -> concat_a/2
  reinterp_b_re/1 -> concat_b/1
  reinterp_b_im/1 -> concat_b/2
  reinterp_a_re/1 -> concat_a/1
  cast_c_re/1 -> c_re/1
  cast_c_im/1 -> c_im/1
